simulink model "ekf_navigation"  (R2026a)
settings: Solver=FixedStepDiscrete  StopTime=Tend  FixedStep=Ts
values from neighbouring files (symbols this model uses):
  P0 = [0.0025 0 0 0 0 0 0 0.0025 0 0 0 0 ... (36 elements, 6x6)]    [ekf_params.mat]    (also in main_kalman.m = diag([0.05^2, 0.05^2, 0.05^2, 0.01^2, 0.01^2, 0.005^2]))
  pv = [p.Ts; p.L; p.tau_v; p.tau_d; p.k_delta; p.k_g;        p.q(:); p.R_v; p.R_g; p.R_xy; p.R_psi]    [ekf_param_vector.m]    (also in ekf_params.mat = [0.02 0.324 0.278090044723 0.0994912869535 1.38661760638 1.0; main_kalman.m = ekf_param_vector(p))
  Ts = D.Ts    [ekf_identify.m]    (also in ekf_params.mat = 0.02; ekf_step.m = pv(1); main_kalman.m = 0.02)
  use_mask = [1 1 1]    [build_ekf_simulink.m]
  x0 = [2.6510733511 -0.283295949553 -0.383685561197 0 0 0.000108295552262]    [ekf_params.mat]    (also in main_kalman.m = [D.x_pf(D.k0); D.y_pf(D.k0); D.psi_pf(D.k0); 0; 0; p.k_g * p)
settings Model: ExtModeTrigDuration=10000  Creator=danielappel  LastModifiedBy=danielappel

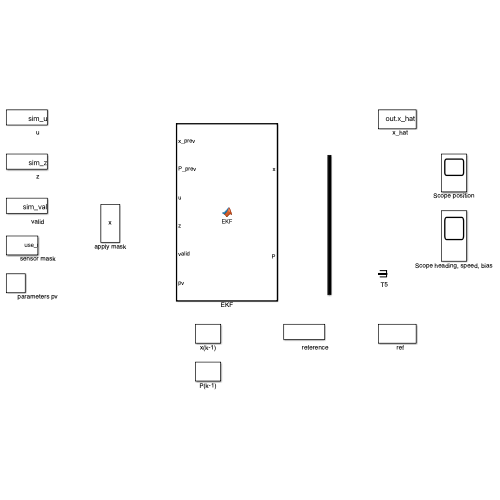
[thumbnail: Simulink's stored preview of the top-level diagram]
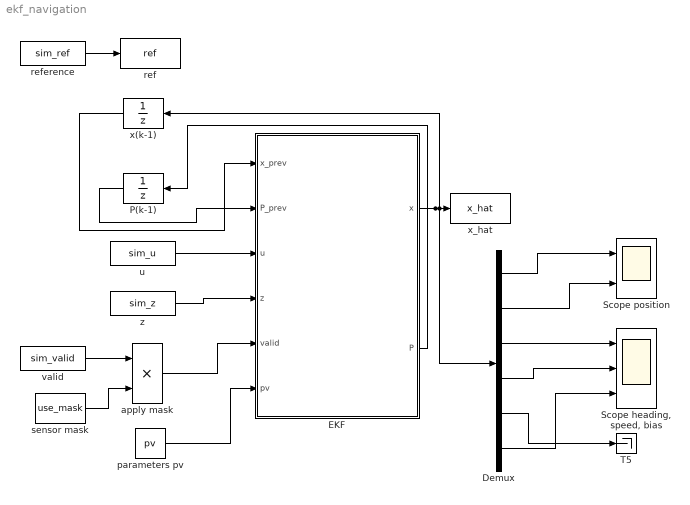
== system ekf_navigation ==
  Demux : Demux  Outputs=6
  EKF : MATLAB Function  TreatAsAtomicUnit=on
  P(k-1) : UnitDelay  InitialCondition=P0  SampleTime=Ts
  "Scope heading, speed, bias" : Scope  NumInputPorts=3
  Scope position : Scope  NumInputPorts=2
  T5 : Terminator
  apply mask : Product
  parameters pv : Constant  Value=pv  SampleTime=Ts
  ref : ToWorkspace  VariableName=ref  SampleTime=Ts
  reference : FromWorkspace  VariableName=sim_ref  SampleTime=Ts  Interpolate=off  OutputAfterFinalValue=Holding final value
  sensor mask : Constant  Value=use_mask  SampleTime=Ts
  u : FromWorkspace  VariableName=sim_u  SampleTime=Ts  Interpolate=off  OutputAfterFinalValue=Holding final value
  valid : FromWorkspace  VariableName=sim_valid  SampleTime=Ts  Interpolate=off  OutputAfterFinalValue=Holding final value
  x(k-1) : UnitDelay  InitialCondition=x0  SampleTime=Ts
  x_hat : ToWorkspace  VariableName=x_hat  SampleTime=Ts
  z : FromWorkspace  VariableName=sim_z  SampleTime=Ts  Interpolate=off  OutputAfterFinalValue=Holding final value
  wires:
  Demux/6 -> "Scope heading, speed, bias"/3
  Demux/5 -> T5/1
  Demux/1 -> Scope position/1
  Demux/4 -> "Scope heading, speed, bias"/2
  parameters pv/1 -> EKF/6(pv)
  Demux/2 -> Scope position/2
  apply mask/1 -> EKF/5(valid)
  EKF/1(x) -> Demux/1, x(k-1)/1, x_hat/1
  z/1 -> EKF/4(z)
  u/1 -> EKF/3(u)
  EKF/2(P) -> P(k-1)/1
  reference/1 -> ref/1
  Demux/3 -> "Scope heading, speed, bias"/1
  x(k-1)/1 -> EKF/1(x_prev)
  sensor mask/1 -> apply mask/2
  P(k-1)/1 -> EKF/2(P_prev)
  valid/1 -> apply mask/1

== matlab function ekf_navigation/EKF ==
  data: x_prev input; P_prev input; u input; x output size=[6 1]; z input; valid input; pv input; P output size=[6 6]
function [x, P] = EKF(x_prev, P_prev, u, z, valid, pv)
%#codegen
% Discrete EKF: prediction with u(k), correction with available measurements
[x, P] = ekf_step(x_prev, P_prev, u, z, valid, pv);
